simulink model "aero2_professor_motor_saturation_experiment"  (R2024b)
settings: Solver=ode1  StartTime=0.0  StopTime=5  FixedStep=0.002  RelTol=1e-3
model workspace (MAT data in the model file):
  Command = [0  0; 0.1  1000; 2  1000; 2.002  0; 5  0]
  ki_PI_motor = 1.84164606325
  kp_PI_motor = 0.216370391856
  kw_PI_motor = 10.85985
settings Model: Creator=matiasgarcia  LastModifiedBy=matiasgarcia

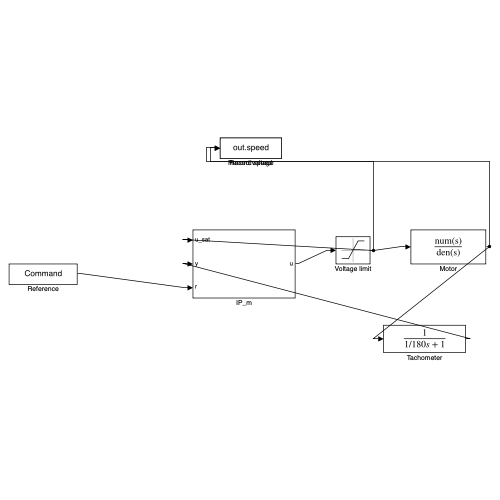
[thumbnail: Simulink's stored preview of the top-level diagram]
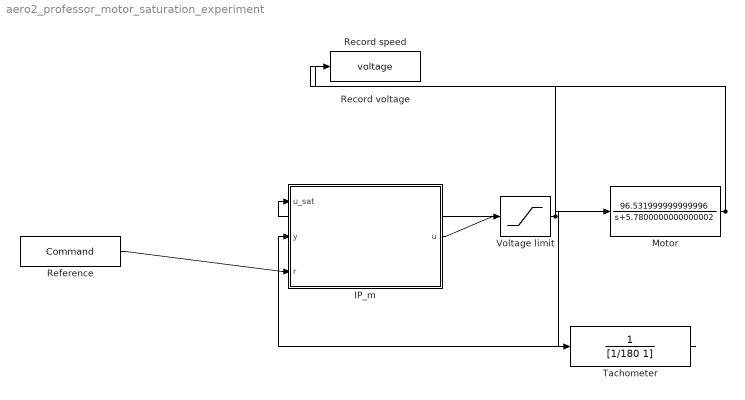
== system aero2_professor_motor_saturation_experiment ==
  IP_m : Subsystem
  Motor : TransferFcn  Numerator=96.531999999999996  Denominator=[1 5.7800000000000002]
  Record speed : ToWorkspace  VariableName=speed  SaveFormat=Timeseries  SampleTime=-1
  Record voltage : ToWorkspace  VariableName=voltage  SaveFormat=Timeseries  SampleTime=-1
  Reference : FromWorkspace  VariableName=Command  Interpolate=off  OutputAfterFinalValue=Holding final value
  Tachometer : TransferFcn  Numerator=1  Denominator=[1/180 1]
  Voltage limit : Saturate  UpperLimit=24  LowerLimit=-24
  wires:
  Reference/1 -> IP_m/3(r)
  IP_m/1(u) -> Voltage limit/1
  Voltage limit/1 -> Motor/1, IP_m/1(u_sat), Record voltage/1
  Motor/1 -> Tachometer/1, Record speed/1
  Tachometer/1 -> IP_m/2(y)

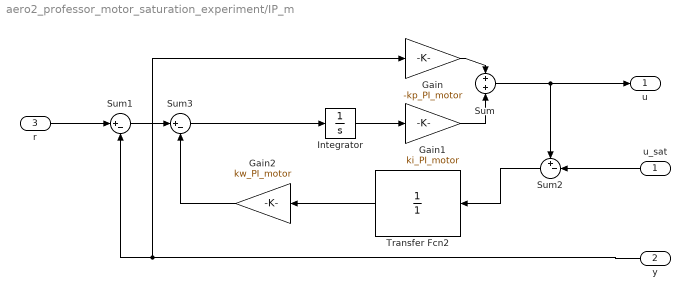
== system aero2_professor_motor_saturation_experiment/IP_m ==
  u_sat : Inport
  y : Inport  Port=2
  r : Inport  Port=3
  Gain : Gain  Gain=-kp_PI_motor
  Gain1 : Gain  Gain=ki_PI_motor
  Gain2 : Gain  Gain=kw_PI_motor
  Integrator : Integrator
  Sum : Sum  Inputs=+|+
  Sum1 : Sum  Inputs=|+-
  Sum2 : Sum  Inputs=+-|
  Sum3 : Sum  Inputs=|+-
  Transfer Fcn2 : TransferFcn  Numerator=1  Denominator=1
  u : Outport
  wires:
  u_sat/1 -> Sum2/2
  r/1 -> Sum1/1
  Sum3/1 -> Integrator/1
  Gain2/1 -> Sum3/2
  Transfer Fcn2/1 -> Gain2/1
  Sum1/1 -> Sum3/1
  Gain1/1 -> Sum/2
  Sum2/1 -> Transfer Fcn2/1
  y/1 -> Sum1/2, Gain/1
  Sum/1 -> Sum2/1, u/1
  Gain/1 -> Sum/1
  Integrator/1 -> Gain1/1
